simulink model "Battery_CCCV_chrging"  (R2024b)
settings: Solver=VariableStepAuto  StartTime=0.0  StopTime=10.0  RelTol=1e-3
undefined symbols (not defined in the file): Ion, Lithium
libraries: spsIdealSwitchLib x2, spsBatteryLib x1, spsControlledCurrentSourceLib x1, spsControlledVoltageSourceLib x1, spsDiodeLib x1, spsSeriesRLCBranchLib x1, spspowerguiLib x1
settings Model: Creator=SUDHAK1  LastModifiedBy=SUDHAK1

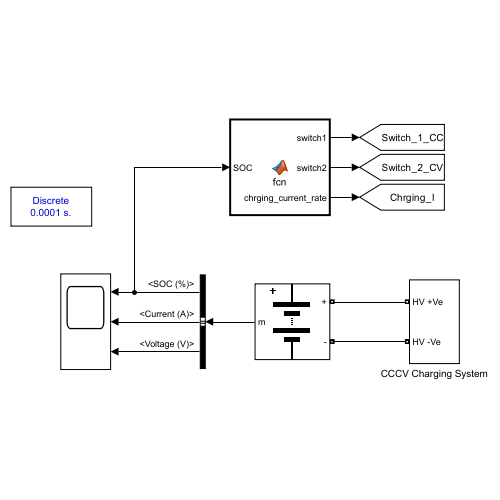
[thumbnail: Simulink's stored preview of the top-level diagram]
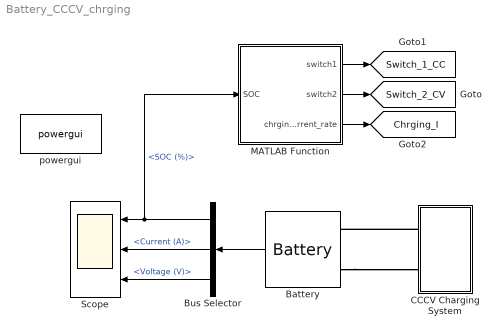
== system Battery_CCCV_chrging ==
  Battery : spsBatteryLib/Battery  BatType=Lithium-Ion  NomV=3.3  NomQ=2.3  SOC=77  Batt_Tr=30  PresetModel=on  MaxQ=2.3  MinV=2.475  FullV=3.8412  Dis_rate=1  R=0.014348  Normal_OP=2.08  expZone="[3.5653       0.113]"
  Bus Selector : BusSelector  OutputSignals=SOC (%),Current (A),Voltage (V)
  CCCV Charging System : Subsystem
  MATLAB Function : MATLAB Function  TreatAsAtomicUnit=on
  Scope : Scope  NumInputPorts=3
  powergui : spspowerguiLib/powergui  Priority=1  SimulationMode=Discrete  SampleTime=1e-4  frequency=60  Iterations=50  frequencyindice=0  Pbase=100e6  ErrMax=1e-4  UnitsV=kV  UnitsW=MW  buscounter=0  FunctionMessages=off  echomessages=off  EnableUseOfTLC=off  CurrentSourceSwitches=off  DisableSnubberDevices=off  DisableRonSwitches=off  DisableVfSwitches=off  DisplayEquations=off  AutomaticDiscreteSolvers=off  SolverType=Tustin/Backward Euler (TBE)  Interpol=off  ExternalGateDelay=off  methode=off  Ts=100  x0status=blocks  SPID=on  SwTol=0  HookPort=off  NonlinearTolerance=1e-4  nMaxIteration=100  ContinueOnMaxIteration=off  RestoreLinks=warning  ResistiveCurrentMeasurement=off  Frange=[0:2:500]  Ylog=off  Xlog=on  ShowGrid=off  save=off  variable=ZData  structure=0  ZoomFFT=off  StartTime=0.0  cycles=1  DisplayStyle=1  fundamental=60  FreqAxis=off  MaxFrequency=1000  frequencyindicesteady=1  RmsSteady=1  display=off
  tag scope: Chrging_I=global, Switch_1_CC=global, Switch_2_CV=global
  wires:
  Battery/1 -> Bus Selector/1
  Bus Selector/2 -> Scope/2  "<Current (A)>"
  Bus Selector/1 -> MATLAB Function/1(SOC), Scope/1  "<SOC (%)>"
  Bus Selector/3 -> Scope/3  "<Voltage (V)>"
  MATLAB Function/1(switch1) -> [Switch_1_CC]
  MATLAB Function/2(switch2) -> [Switch_2_CV]
  MATLAB Function/3(chrging_current_rate) -> [Chrging_I]
  connections:
  CCCV Charging System/LConn1 -- Battery/LConn1
  Battery/LConn2 -- CCCV Charging System/LConn2

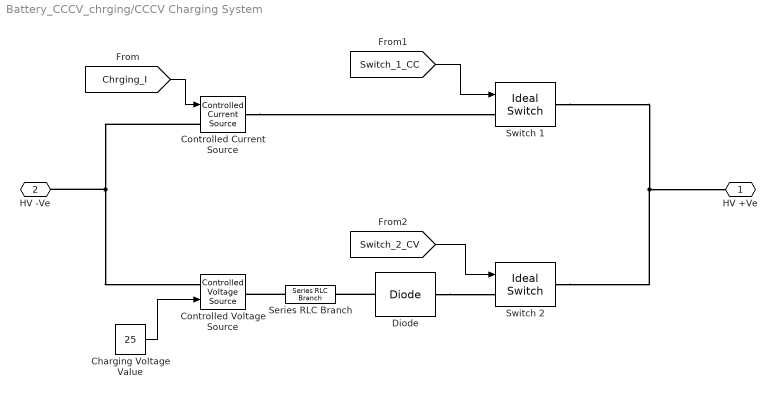
== system Battery_CCCV_chrging/CCCV Charging System ==
  Charging Voltage Value : Constant  Value=25
  Controlled Current Source : spsControlledCurrentSourceLib/Controlled Current Source  Initialize=on  Source_Type=AC  Amplitude=0  Phase=0  Frequency=0  Measurements=None
  Controlled Voltage Source : spsControlledVoltageSourceLib/Controlled Voltage Source  Initialize=on  Source_Type=AC  Amplitude=0  Phase=0  Frequency=0  Measurements=None
  Diode : spsDiodeLib/Diode  Ron=1e-6  Lon=0  Vf=0.8  IC=0  UseSnubber=0  Rs=500  Cs=250e-9  Measurements=off
  Series RLC Branch : spsSeriesRLCBranchLib/Series RLC Branch  LConnTagsString=__new0  RConnTagsString=__new0  BranchType=R  Resistance=1e-3  Inductance=1e-3  SetiL0=off  InitialCurrent=0  Capacitance=1e-6  Setx0=off  InitialVoltage=0  Measurements=None
  Switch 1 : spsIdealSwitchLib/Ideal Switch  Ron=1e-6  Lon=0  IC=0  Rs=1e5  Cs=inf  Measurements=off
  Switch 2 : spsIdealSwitchLib/Ideal Switch  Ron=1e-6  Lon=0  IC=0  Rs=1e5  Cs=inf  Measurements=off
  HV +Ve : PMIOPort  Side=Left
  HV -Ve : PMIOPort  Port=2  Side=Left
  wires:
  Charging Voltage Value/1 -> Controlled Voltage Source/1
  [Switch_1_CC] -> Switch 1/1
  [Switch_2_CV] -> Switch 2/1
  [Chrging_I] -> Controlled Current Source/1
  connections:
  Switch 2/RConn1 -- Switch 1/RConn1 -- HV +Ve/RConn1
  Diode/RConn1 -- Switch 2/LConn1
  Diode/LConn1 -- Series RLC Branch/RConn1
  Series RLC Branch/LConn1 -- Controlled Voltage Source/RConn1
  Controlled Current Source/RConn1 -- Switch 1/LConn1
  Controlled Current Source/LConn1 -- Controlled Voltage Source/LConn1 -- HV -Ve/RConn1

== matlab function Battery_CCCV_chrging/MATLAB Function ==
  data: SOC input; switch1 output; switch2 output; chrging_current_rate output
function [switch1,switch2,chrging_current_rate] = fcn(SOC)

chrging_current_rate=0; % 0Amps initially : Constant current input value

if( (SOC==0) || (SOC <=80))
    switch1=1;
    switch2=0;
    chrging_current_rate=2; % current rate 2 Amps
else
    switch1=0;
    switch2=1;
end
